simulink model "Bossi_Emanuele_EE460S3D_R99"  (R2025a)
settings: Solver=FixedStepDiscrete  StartTime=0.0  StopTime=120  FixedStep=dt0  RelTol=1e-3  EnableMultiTasking=on
PostLoadFcn:
  | %Set the size for the model
  | set_param(gcs,'Location',[10 10 1270 970])
  | %Set the zoom factor for the model
  | set_param(gcs,'ZoomFactor','100')
InitFcn:
  | tic
  | Bossi_Emanuele_EE460_Final
  | INIT_S3D_01
StartFcn:
  | tend0=toc;
  | tic;
StopFcn:
  | tend=toc;
  | disp(['Simulation time = ' num2str(tout(end)) ' sec'])
  | disp(['Real time = ' num2str(tend) ' sec'])
  | title('DONE')
  | SCORE=round((max(0,120-tout(end)-tend0))*4+10*(40-FuelBurned)+sum(100*double(PDONE)-100*double(PDONE<.5)));
  | PlotS3D(PlotInput);
  | text(15,22,['S: ' num2str(SCORE)]);
  | % Reset color scheme back to normal defaults
  | figure()
  | blkwhitebg('w');
  | close
values from neighbouring files (symbols this model uses):
  A_obs = [ 0  1  0  0  0  0 ... (first row only)    [Bossi_Emanuele_EE460_Final.m]
  B_obs = [ 0     0     0 ... (first row only)    [Bossi_Emanuele_EE460_Final.m]
  C_obs = [ 1 0 0 0 0 0 ... (first row only)    [Bossi_Emanuele_EE460_Final.m]
  d2r = pi/180    (= 0.0174532925199)    [INIT_S3D_01.m]
  D_obs = [ 0     0     0 ... (first row only)    [Bossi_Emanuele_EE460_Final.m]
  dt = 0.01    [INIT_S3D_01.m]
  dt0 = 0.001    [INIT_S3D_01.m]
  fr = 100    [INIT_S3D_01.m]
  G = [1,  1, -1, -1,  0,  0,  0,  0 ... (first row only)    [Bossi_Emanuele_EE460_Final.m]
  G_obs = eye(6)    [Bossi_Emanuele_EE460_Final.m]
  HM_S = 250    [INIT_S3D_01.m]
  HM_U = 500    [INIT_S3D_01.m]
  J = Jbase+JC0+JF+M*(Xcg^2+Ycg^2)    [INIT_S3D_01.m]
  Jbase = JC1+4*Ja+2*Ma*da^2+2*Ma*db^2    [INIT_S3D_01.m]
  JC0 = MC0/2    (= 10.2101761242)    [INIT_S3D_01.m]
  Kdtheta = 2 * zeta_th * wn_th * J_eff    [Bossi_Emanuele_EE460_Final.m]
  Kdtheta_fail = 2 * zeta_th_fail * wn_th_fail * J_eff    [Bossi_Emanuele_EE460_Final.m]
  Kdx = 2 * zeta_xy * wn_xy * M_eff    [Bossi_Emanuele_EE460_Final.m]
  Kdx_fail = 2 * zeta_xy_fail * wn_xy_fail * M_eff    [Bossi_Emanuele_EE460_Final.m]
  Kdy = 2 * zeta_xy * wn_xy * M_eff    [Bossi_Emanuele_EE460_Final.m]
  Kdy_fail = 2 * zeta_xy_fail * wn_xy_fail * M_eff    [Bossi_Emanuele_EE460_Final.m]
  Kptheta = J_eff * wn_th^2    [Bossi_Emanuele_EE460_Final.m]
  Kptheta_fail = J_eff * wn_th_fail^2    [Bossi_Emanuele_EE460_Final.m]
  Kpx = M_eff * wn_xy^2    [Bossi_Emanuele_EE460_Final.m]
  Kpx_fail = M_eff * wn_xy_fail^2    [Bossi_Emanuele_EE460_Final.m]
  Kpy = M_eff * wn_xy^2    [Bossi_Emanuele_EE460_Final.m]
  Kpy_fail = M_eff * wn_xy_fail^2    [Bossi_Emanuele_EE460_Final.m]
  L13 = sqrt(10)    [INIT_S3D_01.m]
  L24 = sqrt(6.25)    [INIT_S3D_01.m]
  LVL = LVL12    [INIT_S3D_01.m]
  M = MC+M1+M2+M3+M4+4*Ma    [INIT_S3D_01.m]
  M1 = LVL.M1    [INIT_S3D_01.m]
  M2 = LVL.M2    [INIT_S3D_01.m]
  M3 = LVL.M3    [INIT_S3D_01.m]
  M4 = LVL.M4    [INIT_S3D_01.m]
  max_qddot = [max_qddot_x; max_qddot_y; max_qddot_theta]    [Bossi_Emanuele_EE460_Final.m]
  mdti = (1/300)    (= 0.00333333333333)    [INIT_S3D_01.m]
  P = [1  1 -1 -1  0  0  0  0 ... (first row only)    [Bossi_Emanuele_EE460_Final.m]
  Pdata = [LVL.P1 LVL.P2 LVL.P3 LVL.P4]    [INIT_S3D_01.m]    (also in PlotS3D.m = R*[xt1;yt1+[0 3*tt*TV(idx-13)*TSIG(idx-13) 0]])
  PTvec = [Pdata(:,1);Pdata(:,2);Pdata(:,3);Pdata(:,4) ... (first row only)    [INIT_S3D_01.m]
  Q_obs = eye(6)    [Bossi_Emanuele_EE460_Final.m]
  r2d = 180/pi    (= 57.2957795131)    [INIT_S3D_01.m]
  r_bang = 0.5    [Bossi_Emanuele_EE460_Final.m]
  Sconfig = 1    [Bossi_Emanuele_EE460_Final.m]
  SLIM = [-100 100 ... (first row only)    [INIT_S3D_01.m]
  SQ = [.005 .01 .004 .005 .01 .004 .02 .01 .4]'    [INIT_S3D_01.m]
  SSF = 1./SQ    [INIT_S3D_01.m]
  tau = 0.5    [Bossi_Emanuele_EE460_Final.m]
  TOLdata = [LVL.P1tol LVL.P2tol LVL.P3tol LVL.P4tol]    [INIT_S3D_01.m]
  ULIM = [[Umin Umax];0 0;0 0]    [INIT_S3D_01.m]
undefined symbols (not defined in the file or in its folder): den_lp, den_lp2, DiscIntNeverNeededParam, dt1_bang_3, dt2_bang_3, dtc_bang_3, num_lp, num_lp2, q0_1
libraries: simulink x87, matrix_library x4, sl3dlib x1, aerolibutil x1, aerolibanimutils x1
(part 3 of 8)

== system Bossi_Emanuele_EE460S3D_R99/S3D_Plant/Sensors/ConvertINT16 ==
  SDouble : Inport
  Bus Creator : BusCreator  Inputs=9
  Data Type Conversion{,1..8} (9 alike) : DataTypeConversion  OutDataTypeStr=int16  SampleTime=dt0  SaturateOnIntegerOverflow=off  RndMeth=Floor
  Demux : Demux  Outputs=9
  INT16 : Outport
  wires:
  Data Type Conversion8/1 -> Bus Creator/9  "Sensor9"
  Data Type Conversion7/1 -> Bus Creator/8  "Sensor8"
  Data Type Conversion6/1 -> Bus Creator/7  "Sensor7"
  Data Type Conversion5/1 -> Bus Creator/6  "Sensor6"
  Data Type Conversion4/1 -> Bus Creator/5  "Sensor5"
  Data Type Conversion3/1 -> Bus Creator/4  "Sensor4"
  Data Type Conversion2/1 -> Bus Creator/3  "Sensor3"
  Demux/5 -> Data Type Conversion4/1
  Demux/3 -> Data Type Conversion2/1
  Demux/6 -> Data Type Conversion5/1
  Demux/4 -> Data Type Conversion3/1
  Demux/9 -> Data Type Conversion8/1
  Demux/7 -> Data Type Conversion6/1
  Demux/8 -> Data Type Conversion7/1
  SDouble/1 -> Demux/1
  Data Type Conversion1/1 -> Bus Creator/2  "Sensor2"
  Bus Creator/1 -> INT16/1  "INT16"
  Demux/1 -> Data Type Conversion/1
  Demux/2 -> Data Type Conversion1/1
  Data Type Conversion/1 -> Bus Creator/1  "Sensor1"

== system Bossi_Emanuele_EE460S3D_R99/S3D_Plant/Sensors/HealthMonitoring ==
  SensorValues : Inport
  Bus Creator1 : BusCreator  Inputs=18
  Bus Selector1 : BusSelector  OutputSignals=Sensor1,Sensor2,Sensor3,Sensor4,Sensor5,Sensor6,Sensor7,Sensor8,Sensor9
  Bus Selector2 : BusSelector  OutputSignals=Sensor1,Sensor2,Sensor3,Sensor4,Sensor5,Sensor6,Sensor7,Sensor8,Sensor9
  Subsystem : Subsystem
  Subsystem1 : Subsystem
  Subsystem2 : Subsystem
  Subsystem3 : Subsystem
  Subsystem4 : Subsystem
  Subsystem5 : Subsystem
  Subsystem6 : Subsystem
  Subsystem7 : Subsystem
  Subsystem8 : Subsystem
  Sensors : Outport
  wires:
  Bus Creator1/1 -> Sensors/1  "Sensors"
  Bus Selector2/4 -> Bus Creator1/4  "<Sensor4>"
  Bus Selector2/8 -> Bus Creator1/8  "<Sensor8>"
  Bus Selector2/6 -> Bus Creator1/6  "<Sensor6>"
  Bus Selector2/5 -> Bus Creator1/5  "<Sensor5>"
  Bus Selector2/3 -> Bus Creator1/3  "<Sensor3>"
  Bus Selector2/9 -> Bus Creator1/9  "<Sensor9>"
  Bus Selector2/2 -> Bus Creator1/2  "<Sensor2>"
  Bus Selector2/1 -> Bus Creator1/1  "<Sensor1>"
  Bus Selector2/7 -> Bus Creator1/7  "<Sensor7>"
  SensorValues/1 -> Bus Selector1/1, Bus Selector2/1
  Subsystem/1(Out1) -> Bus Creator1/10  "S1fail"
  Bus Selector1/8 -> Subsystem7/1(In1)  "<Sensor8>"
  Bus Selector1/3 -> Subsystem2/1(In1)  "<Sensor3>"
  Bus Selector1/7 -> Subsystem6/1(In1)  "<Sensor7>"
  Bus Selector1/2 -> Subsystem1/1(In1)  "<Sensor2>"
  Subsystem2/1(Out1) -> Bus Creator1/12  "S3fail"
  Subsystem1/1(Out1) -> Bus Creator1/11  "S2fail"
  Bus Selector1/6 -> Subsystem5/1(In1)  "<Sensor6>"
  Subsystem3/1(Out1) -> Bus Creator1/13  "S4fail"
  Bus Selector1/4 -> Subsystem3/1(In1)  "<Sensor4>"
  Bus Selector1/5 -> Subsystem4/1(In1)  "<Sensor5>"
  Bus Selector1/9 -> Subsystem8/1(In1)  "<Sensor9>"
  Subsystem5/1(Out1) -> Bus Creator1/15  "S6fail"
  Subsystem4/1(Out1) -> Bus Creator1/14  "S5fail"
  Subsystem6/1(Out1) -> Bus Creator1/16  "S7fail"
  Subsystem8/1(Out1) -> Bus Creator1/18  "S9fail"
  Subsystem7/1(Out1) -> Bus Creator1/17  "S8fail"
  Bus Selector1/1 -> Subsystem/1(In1)  "<Sensor1>"

== system Bossi_Emanuele_EE460S3D_R99/S3D_Plant/ThrusterValues/FailModes ==
  Ucmd : Inport
  MP : Inport  Port=2
  Bus Creator : BusCreator  Inputs=10
  Ufail1 : Subsystem  mask{Udx=1, Tank=1}
      mask prompts: Udx "Input Index of U (1-8)"; Tank "Input Fuel Tank (1-4)"
  Ufail10 : Subsystem  mask{Udx=10, Tank=1}
      mask prompts: Udx "Input Index of U (1-8)"; Tank "Input Fuel Tank (1-4)"
  Ufail2 : Subsystem  mask{Udx=2, Tank=2}
      mask prompts: Udx "Input Index of U (1-8)"; Tank "Input Fuel Tank (1-4)"
  Ufail3 : Subsystem  mask{Udx=3, Tank=3}
      mask prompts: Udx "Input Index of U (1-8)"; Tank "Input Fuel Tank (1-4)"
  Ufail4 : Subsystem  mask{Udx=4, Tank=4}
      mask prompts: Udx "Input Index of U (1-8)"; Tank "Input Fuel Tank (1-4)"
  Ufail5 : Subsystem  mask{Udx=5, Tank=1}
      mask prompts: Udx "Input Index of U (1-8)"; Tank "Input Fuel Tank (1-4)"
  Ufail6 : Subsystem  mask{Udx=6, Tank=2}
      mask prompts: Udx "Input Index of U (1-8)"; Tank "Input Fuel Tank (1-4)"
  Ufail7 : Subsystem  mask{Udx=7, Tank=3}
      mask prompts: Udx "Input Index of U (1-8)"; Tank "Input Fuel Tank (1-4)"
  Ufail8 : Subsystem  mask{Udx=8, Tank=4}
      mask prompts: Udx "Input Index of U (1-8)"; Tank "Input Fuel Tank (1-4)"
  Ufail9 : Subsystem  mask{Udx=9, Tank=1}
      mask prompts: Udx "Input Index of U (1-8)"; Tank "Input Fuel Tank (1-4)"
  U : Outport
  wires:
  Bus Creator/1 -> U/1  "U"
  Ufail7/1(Uout) -> Bus Creator/7  "U7"
  Ufail6/1(Uout) -> Bus Creator/6  "U6"
  Ufail8/1(Uout) -> Bus Creator/8  "U8"
  Ufail9/1(Uout) -> Bus Creator/9  "U9"
  Ufail10/1(Uout) -> Bus Creator/10  "U10"
  Ufail5/1(Uout) -> Bus Creator/5  "U5"
  Ufail4/1(Uout) -> Bus Creator/4  "U4"
  Ufail3/1(Uout) -> Bus Creator/3  "U3"
  Ufail2/1(Uout) -> Bus Creator/2  "U2"
  Ufail1/1(Uout) -> Bus Creator/1  "U1"
  MP/1 -> Ufail1/2(MP), Ufail3/2(MP), Ufail4/2(MP), Ufail8/2(MP), Ufail7/2(MP), Ufail6/2(MP), Ufail5/2(MP), Ufail2/2(MP)
  Ucmd/1 -> Ufail1/1(Uin), Ufail4/1(Uin), Ufail9/1(Uin), Ufail10/1(Uin), Ufail8/1(Uin), Ufail7/1(Uin), Ufail6/1(Uin), Ufail5/1(Uin), Ufail3/1(Uin), Ufail2/1(Uin)

== system Bossi_Emanuele_EE460S3D_R99/S3D_Plant/ThrusterValues/HealthMonitoring ==
  Uvalues : Inport
  UCMD : Inport  Port=2
  Bus Creator2 : BusCreator  Inputs=20
  Bus Selector10 : BusSelector  OutputSignals=U1,U2,U3,U4,U5,U6,U7,U8,U9,U10
  Bus Selector11 : BusSelector  OutputSignals=U1fail,U2fail,U3fail,U4fail,U5fail,U6fail,U7fail,U8fail,U9fail,U10fail
  DetectFailures : Subsystem
  U : Outport
  wires:
  Bus Selector10/1 -> Bus Creator2/1  "<U1>"
  Bus Selector10/2 -> Bus Creator2/2  "<U2>"
  Bus Selector10/9 -> Bus Creator2/9  "<U9>"
  Bus Selector10/5 -> Bus Creator2/5  "<U5>"
  Bus Selector10/3 -> Bus Creator2/3  "<U3>"
  Bus Selector10/6 -> Bus Creator2/6  "<U6>"
  Bus Selector10/7 -> Bus Creator2/7  "<U7>"
  Bus Selector10/8 -> Bus Creator2/8  "<U8>"
  Bus Selector10/4 -> Bus Creator2/4  "<U4>"
  Bus Selector10/10 -> Bus Creator2/10  "<U10>"
  Bus Creator2/1 -> U/1  "U"
  Bus Selector11/1 -> Bus Creator2/11  "<U1fail>"
  Bus Selector11/2 -> Bus Creator2/12  "<U2fail>"
  Bus Selector11/3 -> Bus Creator2/13  "<U3fail>"
  Bus Selector11/4 -> Bus Creator2/14  "<U4fail>"
  Bus Selector11/5 -> Bus Creator2/15  "<U5fail>"
  Bus Selector11/6 -> Bus Creator2/16  "<U6fail>"
  Bus Selector11/7 -> Bus Creator2/17  "<U7fail>"
  Bus Selector11/8 -> Bus Creator2/18  "<U8fail>"
  Bus Selector11/9 -> Bus Creator2/19  "<U9fail>"
  Bus Selector11/10 -> Bus Creator2/20  "<U10fail>"
  UCMD/1 -> DetectFailures/2(UCMD)
  Uvalues/1 -> DetectFailures/1(Uvalues), Bus Selector10/1
  DetectFailures/1(Out2) -> Bus Selector11/1

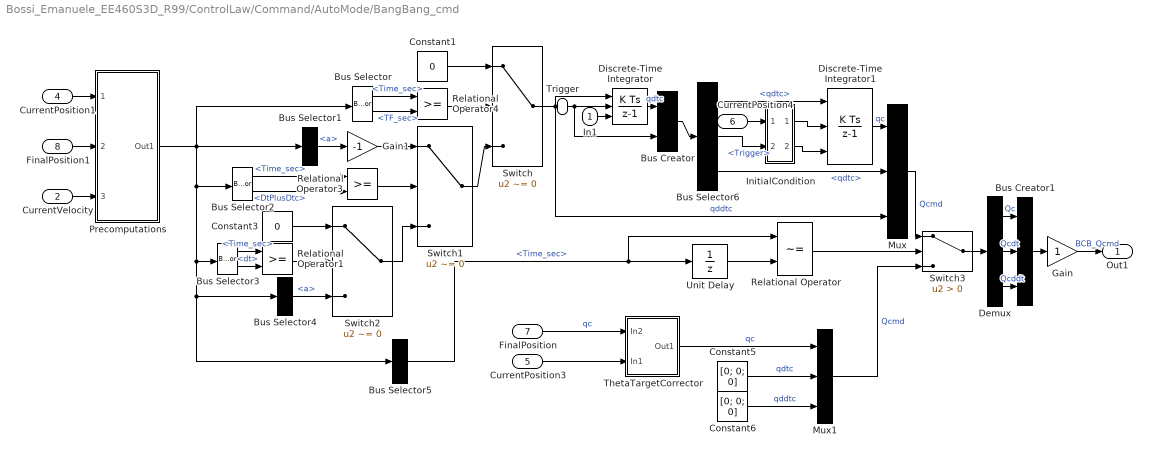
== system Bossi_Emanuele_EE460S3D_R99/ControlLaw/Command/AutoMode/BangBang_cmd ==
  In1 : Inport
  CurrentVelocity : Inport  Port=2
  Trigger : Inport  Port=3
  CurrentPosition1 : Inport  Port=4
  CurrentPosition3 : Inport  Port=5
  CurrentPosition4 : Inport  Port=6
  FinalPosition : Inport  Port=7
  FinalPosition1 : Inport  Port=8
  Bus Creator : BusCreator  Inputs=2
  Bus Creator1 : BusCreator  Inputs=3
  Bus Selector : BusSelector  OutputSignals=Time_sec,TF_sec
  Bus Selector1 : BusSelector  OutputSignals=a
  Bus Selector2 : BusSelector  OutputSignals=Time_sec,DtPlusDtc
  Bus Selector3 : BusSelector  OutputSignals=Time_sec,dt
  Bus Selector4 : BusSelector  OutputSignals=a
  Bus Selector5 : BusSelector  OutputSignals=Time_sec
  Bus Selector6 : BusSelector  OutputSignals=qdtc,Trigger,qdtc
  Constant1 : Constant  Value=0
  Constant3 : Constant  Value=0
  Constant5 : Constant  Value=[0; 0; 0]
  Constant6 : Constant  Value=[0; 0; 0]
  Demux : Demux  Outputs=3
  Discrete-Time Integrator : DiscreteIntegrator  ExternalReset=rising  InitialConditionSource=external  SampleTime=dt  ICPrevOutput=DiscIntNeverNeededParam  ICPrevScaledInput=DiscIntNeverNeededParam
  Discrete-Time Integrator1 : DiscreteIntegrator  ExternalReset=rising  InitialConditionSource=external  InitialCondition=q0_1  SampleTime=dt  ICPrevOutput=DiscIntNeverNeededParam  ICPrevScaledInput=DiscIntNeverNeededParam
  Gain : Gain
  Gain1 : Gain  Gain=-1
  InitialCondition : Subsystem
  Mux : Mux  Inputs=3
  Mux1 : Mux  Inputs=3
  Precomputations : Subsystem
  Relational Operator : RelationalOperator  Operator=~=  OutDataTypeStr=boolean  RndMeth=Simplest  InputSameDT=off
  Relational Operator1 : RelationalOperator  OutDataTypeStr=boolean  RndMeth=Simplest  InputSameDT=off
  Relational Operator3 : RelationalOperator  OutDataTypeStr=boolean  RndMeth=Simplest  InputSameDT=off
  Relational Operator4 : RelationalOperator  OutDataTypeStr=boolean  RndMeth=Simplest  InputSameDT=off
  Switch : Switch  Criteria=u2 ~= 0  Threshold=dt2_bang_3  SaturateOnIntegerOverflow=off  InputSameDT=off
  Switch1 : Switch  Criteria=u2 ~= 0  Threshold=dtc_bang_3  SaturateOnIntegerOverflow=off  InputSameDT=off
  Switch2 : Switch  Criteria=u2 ~= 0  Threshold=dt1_bang_3  SaturateOnIntegerOverflow=off  InputSameDT=off
  Switch3 : Switch  Criteria=u2 > Threshold  SaturateOnIntegerOverflow=off  InputSameDT=off
  ThetaTargetCorrector : Subsystem
  Unit Delay : UnitDelay  InitialCondition=-dt  SampleTime=dt  HasFrameUpgradeWarning=on
  Out1 : Outport
  wires:
  Bus Creator1/1 -> Gain/1
  Gain/1 -> Out1/1  "BCB_Qcmd"
  Switch3/1 -> Demux/1
  Constant5/1 -> Mux1/2  "qdtc"
  InitialCondition/2(Out2) -> Discrete-Time Integrator1/3
  Constant1/1 -> Switch/1
  Mux1/1 -> Switch3/3  "Qcmd"
  InitialCondition/1(Out1) -> Discrete-Time Integrator1/2
  Demux/1 -> Bus Creator1/1  "Qc"
  Discrete-Time Integrator1/1 -> Mux/1  "qc"
  Trigger/1 -> Discrete-Time Integrator/2, Bus Creator/2
  Unit Delay/1 -> Relational Operator/2
  Constant6/1 -> Mux1/3  "qddtc"
  Demux/2 -> Bus Creator1/2  "Qcdt"
  ThetaTargetCorrector/1(Out1) -> Mux1/1  "qc"
  Demux/3 -> Bus Creator1/3  "Qcddt"
  Switch2/1 -> Switch1/3
  Constant3/1 -> Switch2/1
  Switch/1 -> Mux/3, Discrete-Time Integrator/1  "qddtc"
  CurrentPosition4/1 -> InitialCondition/1(In1)
  FinalPosition/1 -> ThetaTargetCorrector/1(In2)  "qc"
  Bus Selector6/1 -> Discrete-Time Integrator1/1  "<qdtc>"
  Mux/1 -> Switch3/1  "Qcmd"
  Relational Operator/1 -> Switch3/2
  Switch1/1 -> Switch/3
  CurrentPosition3/1 -> ThetaTargetCorrector/2(In1)
  CurrentPosition1/1 -> Precomputations/1(CurrentPosition1)
  FinalPosition1/1 -> Precomputations/2(FinalPosition1)
  Precomputations/1(Out1) -> Bus Selector/1, Bus Selector2/1, Bus Selector5/1, Bus Selector4/1, Bus Selector3/1, Bus Selector1/1
  Gain1/1 -> Switch1/1
  Relational Operator1/1 -> Switch2/2
  Relational Operator3/1 -> Switch1/2
  Relational Operator4/1 -> Switch/2
  Bus Selector1/1 -> Gain1/1  "<a>"
  Bus Selector2/1 -> Relational Operator3/1  "<Time_sec>"
  Bus Selector2/2 -> Relational Operator3/2  "<DtPlusDtc>"
  Bus Selector3/2 -> Relational Operator1/2  "<dt>"
  Bus Selector3/1 -> Relational Operator1/1  "<Time_sec>"
  Bus Selector4/1 -> Switch2/3  "<a>"
  Bus Selector5/1 -> Relational Operator/1, Unit Delay/1  "<Time_sec>"
  Bus Selector/1 -> Relational Operator4/1  "<Time_sec>"
  Bus Selector/2 -> Relational Operator4/2  "<TF_sec>"
  Discrete-Time Integrator/1 -> Bus Creator/1  "qdtc"
  Bus Creator/1 -> Bus Selector6/1
  Bus Selector6/2 -> InitialCondition/2(In2)  "<Trigger>"
  Bus Selector6/3 -> Mux/2  "<qdtc>"
  In1/1 -> Discrete-Time Integrator/3
  CurrentVelocity/1 -> Precomputations/3(CurrentVelocity)

== system Bossi_Emanuele_EE460S3D_R99/ControlLaw/Command/AutoMode/FinalPositionSelector ==
  In2 : Inport
  If : If  IfExpression=u1 < 1.5  ElseIfExpressions=u1 < 2.5,u1 < 3.5
  Merge : Merge  Inputs=4
  Pdata1 : Subsystem  TreatAsAtomicUnit=on
  Pdata2 : Subsystem  TreatAsAtomicUnit=on
  Pdata3 : Subsystem  TreatAsAtomicUnit=on
  Pdata4 : Subsystem  TreatAsAtomicUnit=on
  FinalPosition : Outport
  wires:
  In2/1 -> If/1
  If/1 -> Pdata1/Action
  Pdata1/1(Out1) -> Merge/1
  Pdata2/1(Out1) -> Merge/2
  Pdata3/1(Out1) -> Merge/3
  Pdata4/1(Out1) -> Merge/4
  If/2 -> Pdata2/Action
  If/3 -> Pdata3/Action
  If/4 -> Pdata4/Action
  Merge/1 -> FinalPosition/1  "FinalPosition"

== system Bossi_Emanuele_EE460S3D_R99/ControlLaw/Command/AutoMode/PositionTrigger ==
  In1 : Inport
  Trigger : TriggerPort  VariantControl=(inherit)
  Bus Selector : BusSelector  OutputSignals=Xpos_m,Ypos_m,theta_pos_deg
  Vector Concatenate : Concatenate  NumInputs=3
  CurrentPosition1 : Outport
  wires:
  Bus Selector/1 -> Vector Concatenate/1  "<Xpos_m>"
  In1/1 -> Bus Selector/1
  Bus Selector/2 -> Vector Concatenate/2  "<Ypos_m>"
  Bus Selector/3 -> Vector Concatenate/3  "<theta_pos_deg>"
  Vector Concatenate/1 -> CurrentPosition1/1  "TriggeredPosition"

== system Bossi_Emanuele_EE460S3D_R99/ControlLaw/Command/AutoMode/TriggerCondition ==
  In2 : Inport
  Relational Operator : RelationalOperator  Operator=~=  OutDataTypeStr=boolean  RndMeth=Simplest  InputSameDT=off
  Unit Delay : UnitDelay  SampleTime=dt  HasFrameUpgradeWarning=on
  Trigger : Outport
  wires:
  Relational Operator/1 -> Trigger/1  "Trigger"
  In2/1 -> Relational Operator/1, Unit Delay/1
  Unit Delay/1 -> Relational Operator/2

== system Bossi_Emanuele_EE460S3D_R99/ControlLaw/Command/AutoMode/VelocityTrigger ==
  In1 : Inport
  Trigger : TriggerPort  VariantControl=(inherit)
  Bus Selector : BusSelector  OutputSignals=Xvel_mps,Yvel_mps,theta_vel_degps
  Vector Concatenate : Concatenate  NumInputs=3
  CurrentVelocity : Outport
  wires:
  In1/1 -> Bus Selector/1
  Vector Concatenate/1 -> CurrentVelocity/1  "TriggeredVelocity"
  Bus Selector/1 -> Vector Concatenate/1  "<Xvel_mps>"
  Bus Selector/2 -> Vector Concatenate/2  "<Yvel_mps>"
  Bus Selector/3 -> Vector Concatenate/3  "<theta_vel_degps>"

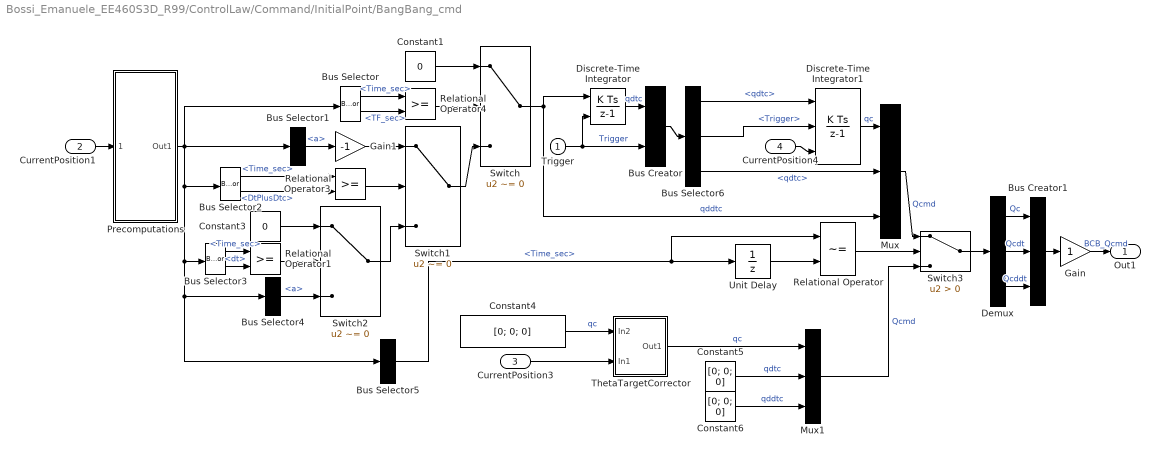
== system Bossi_Emanuele_EE460S3D_R99/ControlLaw/Command/InitialPoint/BangBang_cmd ==
  Trigger : Inport
  CurrentPosition1 : Inport  Port=2
  CurrentPosition3 : Inport  Port=3
  CurrentPosition4 : Inport  Port=4
  Bus Creator : BusCreator  Inputs=2
  Bus Creator1 : BusCreator  Inputs=3
  Bus Selector : BusSelector  OutputSignals=Time_sec,TF_sec
  Bus Selector1 : BusSelector  OutputSignals=a
  Bus Selector2 : BusSelector  OutputSignals=Time_sec,DtPlusDtc
  Bus Selector3 : BusSelector  OutputSignals=Time_sec,dt
  Bus Selector4 : BusSelector  OutputSignals=a
  Bus Selector5 : BusSelector  OutputSignals=Time_sec
  Bus Selector6 : BusSelector  OutputSignals=qdtc,Trigger,qdtc
  Constant1 : Constant  Value=0
  Constant3 : Constant  Value=0
  Constant4 : Constant  Value=[0; 0; 0]  SampleTime=dt
  Constant5 : Constant  Value=[0; 0; 0]
  Constant6 : Constant  Value=[0; 0; 0]
  Demux : Demux  Outputs=3
  Discrete-Time Integrator : DiscreteIntegrator  ExternalReset=rising  SampleTime=dt  ICPrevOutput=DiscIntNeverNeededParam  ICPrevScaledInput=DiscIntNeverNeededParam
  Discrete-Time Integrator1 : DiscreteIntegrator  ExternalReset=rising  InitialConditionSource=external  InitialCondition=q0_1  SampleTime=dt  ICPrevOutput=DiscIntNeverNeededParam  ICPrevScaledInput=DiscIntNeverNeededParam
  Gain : Gain
  Gain1 : Gain  Gain=-1
  Mux : Mux  Inputs=3
  Mux1 : Mux  Inputs=3
  Precomputations : Subsystem
  Relational Operator : RelationalOperator  Operator=~=  OutDataTypeStr=boolean  RndMeth=Simplest  InputSameDT=off
  Relational Operator1 : RelationalOperator  OutDataTypeStr=boolean  RndMeth=Simplest  InputSameDT=off
  Relational Operator3 : RelationalOperator  OutDataTypeStr=boolean  RndMeth=Simplest  InputSameDT=off
  Relational Operator4 : RelationalOperator  OutDataTypeStr=boolean  RndMeth=Simplest  InputSameDT=off
  Switch : Switch  Criteria=u2 ~= 0  Threshold=dt2_bang_3  SaturateOnIntegerOverflow=off  InputSameDT=off
  Switch1 : Switch  Criteria=u2 ~= 0  Threshold=dtc_bang_3  SaturateOnIntegerOverflow=off  InputSameDT=off
  Switch2 : Switch  Criteria=u2 ~= 0  Threshold=dt1_bang_3  SaturateOnIntegerOverflow=off  InputSameDT=off
  Switch3 : Switch  Criteria=u2 > Threshold  SaturateOnIntegerOverflow=off  InputSameDT=off
  ThetaTargetCorrector : Subsystem
  Unit Delay : UnitDelay  InitialCondition=-dt  SampleTime=dt  HasFrameUpgradeWarning=on
  Out1 : Outport
  wires:
  Bus Creator1/1 -> Gain/1
  Gain/1 -> Out1/1  "BCB_Qcmd"
  Switch3/1 -> Demux/1
  Constant5/1 -> Mux1/2  "qdtc"
  Constant1/1 -> Switch/1
  Mux1/1 -> Switch3/3  "Qcmd"
  Demux/1 -> Bus Creator1/1  "Qc"
  Discrete-Time Integrator1/1 -> Mux/1  "qc"
  Unit Delay/1 -> Relational Operator/2
  Constant6/1 -> Mux1/3  "qddtc"
  Demux/2 -> Bus Creator1/2  "Qcdt"
  ThetaTargetCorrector/1(Out1) -> Mux1/1  "qc"
  Demux/3 -> Bus Creator1/3  "Qcddt"
  Switch2/1 -> Switch1/3
  Constant3/1 -> Switch2/1
  Switch/1 -> Mux/3, Discrete-Time Integrator/1  "qddtc"
  CurrentPosition4/1 -> Discrete-Time Integrator1/3
  Constant4/1 -> ThetaTargetCorrector/1(In2)  "qc"
  Bus Selector6/1 -> Discrete-Time Integrator1/1  "<qdtc>"
  Mux/1 -> Switch3/1  "Qcmd"
  Relational Operator/1 -> Switch3/2
  Switch1/1 -> Switch/3
  CurrentPosition3/1 -> ThetaTargetCorrector/2(In1)
  CurrentPosition1/1 -> Precomputations/1(CurrentPosition1)
  Precomputations/1(Out1) -> Bus Selector/1, Bus Selector2/1, Bus Selector5/1, Bus Selector4/1, Bus Selector3/1, Bus Selector1/1
  Gain1/1 -> Switch1/1
  Relational Operator1/1 -> Switch2/2
  Relational Operator3/1 -> Switch1/2
  Relational Operator4/1 -> Switch/2
  Bus Selector1/1 -> Gain1/1  "<a>"
  Bus Selector2/1 -> Relational Operator3/1  "<Time_sec>"
  Bus Selector2/2 -> Relational Operator3/2  "<DtPlusDtc>"
  Bus Selector3/2 -> Relational Operator1/2  "<dt>"
  Bus Selector3/1 -> Relational Operator1/1  "<Time_sec>"
  Bus Selector4/1 -> Switch2/3  "<a>"
  Bus Selector5/1 -> Relational Operator/1, Unit Delay/1  "<Time_sec>"
  Bus Selector/1 -> Relational Operator4/1  "<Time_sec>"
  Bus Selector/2 -> Relational Operator4/2  "<TF_sec>"
  Discrete-Time Integrator/1 -> Bus Creator/1  "qdtc"
  Bus Creator/1 -> Bus Selector6/1
  Bus Selector6/3 -> Mux/2  "<qdtc>"
  Trigger/1 -> Discrete-Time Integrator/2, Bus Creator/2  "Trigger"
  Bus Selector6/2 -> Discrete-Time Integrator1/2  "<Trigger>"

== system Bossi_Emanuele_EE460S3D_R99/ControlLaw/Command/Joystick/Hold ==
  In1 : Inport
  Logical Operator : Logic  Operator=NOT  AllPortsSameDT=off  OutDataTypeStr=boolean
  Logical Operator1 : Logic  AllPortsSameDT=off  OutDataTypeStr=boolean
  Logical Operator2 : Logic  Operator=NOT  AllPortsSameDT=off  OutDataTypeStr=boolean
  Switch : Switch  Criteria=u2 > Threshold  SaturateOnIntegerOverflow=off  InputSameDT=off
  Unit Delay : UnitDelay  SampleTime=-1  HasFrameUpgradeWarning=on
  Unit Delay1 : UnitDelay  SampleTime=dt  HasFrameUpgradeWarning=on
  Unit Delay2 : UnitDelay  SampleTime=dt  HasFrameUpgradeWarning=on
  Out1 : Outport
  wires:
  Logical Operator2/1 -> Switch/1
  Switch/1 -> Out1/1, Unit Delay2/1, Unit Delay1/1  "ManualMode"
  Unit Delay1/1 -> Switch/3
  Unit Delay2/1 -> Logical Operator2/1
  Unit Delay/1 -> Logical Operator/1
  Logical Operator1/1 -> Switch/2  "pressEvent"
  Logical Operator/1 -> Logical Operator1/2  "NOT_prevButton"
  In1/1 -> Unit Delay/1, Logical Operator1/1  "Button"

== system Bossi_Emanuele_EE460S3D_R99/ControlLaw/Command/Joystick/Hold1 ==
  In1 : Inport
  Logical Operator : Logic  Operator=NOT  AllPortsSameDT=off  OutDataTypeStr=boolean
  Logical Operator1 : Logic  AllPortsSameDT=off  OutDataTypeStr=boolean
  Logical Operator2 : Logic  Operator=NOT  AllPortsSameDT=off  OutDataTypeStr=boolean
  Switch : Switch  Criteria=u2 > Threshold  SaturateOnIntegerOverflow=off  InputSameDT=off
  Unit Delay : UnitDelay  SampleTime=-1  HasFrameUpgradeWarning=on
  Unit Delay1 : UnitDelay  SampleTime=dt  HasFrameUpgradeWarning=on
  Unit Delay2 : UnitDelay  SampleTime=dt  HasFrameUpgradeWarning=on
  Out1 : Outport
  wires:
  Logical Operator2/1 -> Switch/1
  Switch/1 -> Out1/1, Unit Delay2/1, Unit Delay1/1  "AutoON"
  Unit Delay1/1 -> Switch/3
  Unit Delay2/1 -> Logical Operator2/1
  Unit Delay/1 -> Logical Operator/1
  Logical Operator1/1 -> Switch/2  "pressEvent"
  Logical Operator/1 -> Logical Operator1/2  "NOT_prevButton"
  In1/1 -> Unit Delay/1, Logical Operator1/1  "Button"

== system Bossi_Emanuele_EE460S3D_R99/ControlLaw/Command/Joystick/MissionNum ==
  In1 : Inport
  In2 : Inport  Port=2
  In3 : Inport  Port=3
  In4 : Inport  Port=4
  Data Type Conversion{,1..3} (4 alike) : DataTypeConversion  OutDataTypeStr=double  SaturateOnIntegerOverflow=off  RndMeth=Floor
  Gain : Gain
  Gain1 : Gain  Gain=2
  Gain2 : Gain  Gain=3
  Gain3 : Gain  Gain=4
  Sum : Sum  Inputs=++++
  Out1 : Outport
  wires:
  In3/1 -> Data Type Conversion2/1
  Gain3/1 -> Sum/4
  Data Type Conversion2/1 -> Gain2/1
  Gain1/1 -> Sum/2
  In4/1 -> Data Type Conversion3/1
  Gain2/1 -> Sum/3
  In2/1 -> Data Type Conversion1/1
  Gain/1 -> Sum/1
  Data Type Conversion3/1 -> Gain3/1
  Data Type Conversion/1 -> Gain/1
  In1/1 -> Data Type Conversion/1
  Data Type Conversion1/1 -> Gain1/1
  Sum/1 -> Out1/1  "MissionNum"

== system Bossi_Emanuele_EE460S3D_R99/ControlLaw/Command/Joystick/PointToGo ==
  Y_IN : Inport
  In1 : Inport  Port=2
  Bus Creator : BusCreator  Inputs=3
  Bus Creator1 : BusCreator  Inputs=4
  Bus Selector : BusSelector  OutputSignals=P1Done,P2Done,P3Done,P4Done
  Bus Selector1 : BusSelector  OutputSignals=UserChoice,MissionNum
  Bus Selector2 : BusSelector  OutputSignals=UserChoice,newSelection
  Bus Selector3 : BusSelector  OutputSignals=hold_active,MissionNum
  Cast To Double : DataTypeConversion  OutDataTypeStr=double  SaturateOnIntegerOverflow=off  RndMeth=Floor
  Compare To Constant : simulink/Logic and Bit Operations/Compare To Constant  relop=<  const=1  OutDataTypeStr=boolean
  Constant : Constant
  Data Type Conversion{,1..3} (4 alike) : DataTypeConversion  OutDataTypeStr=double  SaturateOnIntegerOverflow=off  RndMeth=Floor
  Hold : Subsystem
  Sum : Sum  Inputs=++++
  Sum2 : Sum  Inputs=|++
  Switch : Switch  Criteria=u2 > Threshold  Threshold=0.5  SaturateOnIntegerOverflow=off  InputSameDT=off
  Switch1 : Switch  Criteria=u2 > Threshold  SaturateOnIntegerOverflow=off  InputSameDT=off
  Unit Delay : UnitDelay  InitialCondition=1  SampleTime=dt  HasFrameUpgradeWarning=on
  Out1 : Outport
  wires:
  In1/1 -> Bus Creator/3, Compare To Constant/1
  Bus Selector/1 -> Data Type Conversion/1  "<P1Done>"
  Data Type Conversion1/1 -> Sum/2
  Bus Selector/4 -> Data Type Conversion3/1  "<P4Done>"
  Y_IN/1 -> Bus Selector/1
  Bus Selector/3 -> Data Type Conversion2/1  "<P3Done>"
  Data Type Conversion2/1 -> Sum/3
  Bus Selector/2 -> Data Type Conversion1/1  "<P2Done>"
  Compare To Constant/1 -> Bus Creator/2  "SwitchCondition"
  Data Type Conversion/1 -> Sum/1
  Data Type Conversion3/1 -> Sum/4
  Sum/1 -> Sum2/1
  Sum2/1 -> Bus Creator/1  "MissionNum"
  Constant/1 -> Sum2/2
  Bus Creator/1 -> Bus Selector1/1, Hold/1(In1)  "Trigger"
  Unit Delay/1 -> Switch/3  "UserChoice_latched_prev"
  Switch/1 -> Unit Delay/1, Cast To Double/1  "UserChoice_latched"
  Bus Selector1/1 -> Bus Creator1/1  "<UserChoice>"
  Bus Creator1/1 -> Bus Selector2/1, Bus Selector3/1
  Bus Selector2/1 -> Switch/1  "<UserChoice>"
  Bus Selector2/2 -> Switch/2  "<newSelection>"
  Bus Selector3/1 -> Switch1/2  "<hold_active>"
  Switch1/1 -> Out1/1  "PointToGo"
  Hold/2(Out2) -> Bus Creator1/4
  Hold/1(Out1) -> Bus Creator1/3
  Bus Selector1/2 -> Bus Creator1/2  "<MissionNum>"
  Bus Selector3/2 -> Switch1/3  "<MissionNum>"
  Cast To Double/1 -> Switch1/1

== system Bossi_Emanuele_EE460S3D_R99/ControlLaw/Command/ManualMode/Theta_cmd ==
  In1 : Inport
  In4 : Inport  Port=2
  In3 : Inport  Port=3
  In2 : Inport  Port=4
  In5 : Inport  Port=5
  Bus Creator5 : BusCreator  Inputs=1
  Bus Creator6 : BusCreator  Inputs=1
  Bus Selector5 : BusSelector  OutputSignals=theta_ddot_cmd,theta_ddot_cmd
  Bus Selector6 : BusSelector  OutputSignals=theta_dot_cmd,theta_dot_cmd,theta_dot_cmd
  Constant2 : Constant  Value=3
  Dead Zone2 : DeadZone  LowerValue=-0.05  UpperValue=0.05
  Discrete-Time Integrator4 : DiscreteIntegrator  ExternalReset=either  InitialConditionSource=external  SampleTime=dt  ICPrevOutput=DiscIntNeverNeededParam  ICPrevScaledInput=DiscIntNeverNeededParam
  Discrete-Time Integrator5 : DiscreteIntegrator  ExternalReset=either  InitialConditionSource=external  SampleTime=dt  ICPrevOutput=DiscIntNeverNeededParam  ICPrevScaledInput=DiscIntNeverNeededParam
  Gain : Gain  Gain=-1
  Gain2 : Gain  Gain=20
  Gain5 : Gain  Gain=1/tau
  Math Function2 : Math  Operator=pow
  Saturation : Saturate  UpperLimit=800  LowerLimit=-800
  Sum2 : Sum  Inputs=|-+|
  Out1 : Outport
  Out2 : Outport  Port=2
  Out3 : Outport  Port=3
  wires:
  Discrete-Time Integrator5/1 -> Out1/1  "theta_cmd"
  Bus Selector6/3 -> Out2/1  "<theta_dot_cmd>"
  Bus Selector5/2 -> Out3/1  "<theta_ddot_cmd>"
  Gain5/1 -> Bus Creator5/1  "theta_ddot_cmd"
  In1/1 -> Saturation/1
  Dead Zone2/1 -> Math Function2/1  "u_r_f"
  Constant2/1 -> Math Function2/2
  Bus Creator6/1 -> Bus Selector6/1
  Math Function2/1 -> Gain2/1  "u_r_shaped"
  Bus Selector6/2 -> Discrete-Time Integrator5/1  "<theta_dot_cmd>"
  Bus Selector5/1 -> Discrete-Time Integrator4/1  "<theta_ddot_cmd>"
  Gain2/1 -> Sum2/2  "theta_dot_des"
  Bus Selector6/1 -> Sum2/1  "<theta_dot_cmd>"
  Discrete-Time Integrator4/1 -> Bus Creator6/1  "theta_dot_cmd"
  Sum2/1 -> Gain5/1
  Bus Creator5/1 -> Bus Selector5/1
  Gain/1 -> Dead Zone2/1
  Saturation/1 -> Gain/1
  In3/1 -> Discrete-Time Integrator4/3
  In2/1 -> Discrete-Time Integrator4/2
  In4/1 -> Discrete-Time Integrator5/3
  In5/1 -> Discrete-Time Integrator5/2

== system Bossi_Emanuele_EE460S3D_R99/ControlLaw/Command/ManualMode/X_cmd ==
  In1 : Inport
  In5 : Inport  Port=2
  In3 : Inport  Port=3
  In2 : Inport  Port=4
  In4 : Inport  Port=5
  Bus Creator1 : BusCreator  Inputs=1
  Bus Creator2 : BusCreator  Inputs=1
  Bus Selector1 : BusSelector  OutputSignals=xddot_cmd,xddot_cmd
  Bus Selector2 : BusSelector  OutputSignals=xdot_cmd,xdot_cmd,xdot_cmd
  Constant : Constant  Value=3
  Dead Zone : DeadZone  LowerValue=-0.05  UpperValue=0.05
  Discrete-Time Integrator : DiscreteIntegrator  ExternalReset=either  InitialConditionSource=external  SampleTime=dt  ICPrevOutput=DiscIntNeverNeededParam  ICPrevScaledInput=DiscIntNeverNeededParam
  Discrete-Time Integrator1 : DiscreteIntegrator  ExternalReset=either  InitialConditionSource=external  SampleTime=dt  ICPrevOutput=DiscIntNeverNeededParam  ICPrevScaledInput=DiscIntNeverNeededParam
  Gain : Gain  Gain=4
  Gain3 : Gain  Gain=1/tau
  Math Function : Math  Operator=pow
  Saturation : Saturate  UpperLimit=200  LowerLimit=-200
  Sum : Sum  Inputs=|-+|
  Out1 : Outport
  Out2 : Outport  Port=2
  Out3 : Outport  Port=3
  wires:
  Bus Selector2/2 -> Discrete-Time Integrator1/1  "<xdot_cmd>"
  Discrete-Time Integrator1/1 -> Out1/1  "x_cmd"
  Gain3/1 -> Bus Creator1/1  "xddot_cmd"
  Bus Selector2/3 -> Out2/1  "<xdot_cmd>"
  Bus Selector2/1 -> Sum/1  "<xdot_cmd>"
  Bus Creator2/1 -> Bus Selector2/1
  Dead Zone/1 -> Math Function/1  "u_x_f"
  Bus Selector1/2 -> Out3/1  "<xddot_cmd>"
  Gain/1 -> Sum/2  "xdot_des"
  Bus Creator1/1 -> Bus Selector1/1
  In1/1 -> Saturation/1
  Discrete-Time Integrator/1 -> Bus Creator2/1  "xdot_cmd"
  Sum/1 -> Gain3/1
  Bus Selector1/1 -> Discrete-Time Integrator/1  "<xddot_cmd>"
  Constant/1 -> Math Function/2
  Math Function/1 -> Gain/1  "u_x_shaped"
  Saturation/1 -> Dead Zone/1
  In2/1 -> Discrete-Time Integrator/2
  In3/1 -> Discrete-Time Integrator/3
  In4/1 -> Discrete-Time Integrator1/2
  In5/1 -> Discrete-Time Integrator1/3

== system Bossi_Emanuele_EE460S3D_R99/ControlLaw/Command/ManualMode/Y_cmd ==
  In1 : Inport
  In4 : Inport  Port=2
  In3 : Inport  Port=3
  In2 : Inport  Port=4
  In5 : Inport  Port=5
  Bus Creator3 : BusCreator  Inputs=1
  Bus Creator4 : BusCreator  Inputs=1
  Bus Selector3 : BusSelector  OutputSignals=yddot_cmd,yddot_cmd
  Bus Selector4 : BusSelector  OutputSignals=ydot_cmd,ydot_cmd,ydot_cmd
  Constant1 : Constant  Value=3
  Dead Zone1 : DeadZone  LowerValue=-0.05  UpperValue=0.05
  Discrete-Time Integrator2 : DiscreteIntegrator  ExternalReset=either  InitialConditionSource=external  SampleTime=dt  ICPrevOutput=DiscIntNeverNeededParam  ICPrevScaledInput=DiscIntNeverNeededParam
  Discrete-Time Integrator3 : DiscreteIntegrator  ExternalReset=either  InitialConditionSource=external  SampleTime=dt  ICPrevOutput=DiscIntNeverNeededParam  ICPrevScaledInput=DiscIntNeverNeededParam
  Gain : Gain  Gain=-1
  Gain1 : Gain  Gain=4
  Gain4 : Gain  Gain=1/tau
  Math Function1 : Math  Operator=pow
  Saturation : Saturate  UpperLimit=200  LowerLimit=-200
  Sum1 : Sum  Inputs=|-+|
  Out1 : Outport
  Out2 : Outport  Port=2
  Out3 : Outport  Port=3
  wires:
  Bus Selector4/3 -> Out2/1  "<ydot_cmd>"
  Discrete-Time Integrator3/1 -> Out1/1  "y_cmd"
  Bus Selector3/2 -> Out3/1  "<yddot_cmd>"
  Constant1/1 -> Math Function1/2
  Dead Zone1/1 -> Math Function1/1  "u_y_f"
  In1/1 -> Saturation/1
  Gain4/1 -> Bus Creator3/1  "yddot_cmd"
  Bus Selector3/1 -> Discrete-Time Integrator2/1  "<yddot_cmd>"
  Sum1/1 -> Gain4/1
  Bus Selector4/2 -> Discrete-Time Integrator3/1  "<ydot_cmd>"
  Bus Creator3/1 -> Bus Selector3/1
  Bus Creator4/1 -> Bus Selector4/1
  Discrete-Time Integrator2/1 -> Bus Creator4/1  "ydot_cmd"
  Gain1/1 -> Sum1/2  "ydot_des"
  Math Function1/1 -> Gain1/1  "u_y_shaped"
  Bus Selector4/1 -> Sum1/1  "<ydot_cmd>"
  Gain/1 -> Dead Zone1/1
  Saturation/1 -> Gain/1
  In3/1 -> Discrete-Time Integrator2/3
  In2/1 -> Discrete-Time Integrator2/2
  In4/1 -> Discrete-Time Integrator3/3
  In5/1 -> Discrete-Time Integrator3/2

== system Bossi_Emanuele_EE460S3D_R99/ControlLaw/Command/Trigger1/PositionTrigger ==
  In1 : Inport
  Trigger : TriggerPort  TriggerType=either  VariantControl=(inherit)
  Bus Selector : BusSelector  OutputSignals=Xpos_m,Ypos_m,theta_pos_deg
  Vector Concatenate : Concatenate  NumInputs=3
  CurrentPosition1 : Outport
  wires:
  Bus Selector/1 -> Vector Concatenate/1  "<Xpos_m>"
  In1/1 -> Bus Selector/1
  Bus Selector/2 -> Vector Concatenate/2  "<Ypos_m>"
  Bus Selector/3 -> Vector Concatenate/3  "<theta_pos_deg>"
  Vector Concatenate/1 -> CurrentPosition1/1  "TriggeredPosition"

== system Bossi_Emanuele_EE460S3D_R99/ControlLaw/Command/Trigger1/TriggerCondition ==
  In2 : Inport
  Relational Operator : RelationalOperator  Operator=~=  OutDataTypeStr=boolean  RndMeth=Simplest  InputSameDT=off
  Unit Delay : UnitDelay  SampleTime=dt  HasFrameUpgradeWarning=on
  Trigger : Outport
  wires:
  Relational Operator/1 -> Trigger/1  "Trigger"
  In2/1 -> Relational Operator/1, Unit Delay/1
  Unit Delay/1 -> Relational Operator/2

== system Bossi_Emanuele_EE460S3D_R99/ControlLaw/Command/Trigger2/PositionTrigger ==
  In1 : Inport
  Trigger : TriggerPort  TriggerType=either  VariantControl=(inherit)
  Bus Selector : BusSelector  OutputSignals=Xpos_m,Ypos_m,theta_pos_deg
  Vector Concatenate : Concatenate  NumInputs=3
  CurrentPosition1 : Outport
  wires:
  Bus Selector/1 -> Vector Concatenate/1  "<Xpos_m>"
  In1/1 -> Bus Selector/1
  Bus Selector/2 -> Vector Concatenate/2  "<Ypos_m>"
  Bus Selector/3 -> Vector Concatenate/3  "<theta_pos_deg>"
  Vector Concatenate/1 -> CurrentPosition1/1  "TriggeredPosition"

== system Bossi_Emanuele_EE460S3D_R99/ControlLaw/Command/Trigger2/TriggerCondition ==
  In2 : Inport
  Relational Operator : RelationalOperator  Operator=~=  OutDataTypeStr=boolean  RndMeth=Simplest  InputSameDT=off
  Unit Delay : UnitDelay  SampleTime=dt  HasFrameUpgradeWarning=on
  Trigger : Outport
  wires:
  Relational Operator/1 -> Trigger/1  "Trigger"
  In2/1 -> Relational Operator/1, Unit Delay/1
  Unit Delay/1 -> Relational Operator/2

== system Bossi_Emanuele_EE460S3D_R99/ControlLaw/Command/Trigger2/VelocityTrigger ==
  In1 : Inport
  Trigger : TriggerPort  TriggerType=either  VariantControl=(inherit)
  Bus Selector : BusSelector  OutputSignals=Xvel_mps,Yvel_mps,theta_vel_degps
  Vector Concatenate : Concatenate  NumInputs=3
  CurrentVelocity : Outport
  wires:
  In1/1 -> Bus Selector/1
  Vector Concatenate/1 -> CurrentVelocity/1  "TriggeredVelocity"
  Bus Selector/1 -> Vector Concatenate/1  "<Xvel_mps>"
  Bus Selector/2 -> Vector Concatenate/2  "<Yvel_mps>"
  Bus Selector/3 -> Vector Concatenate/3  "<theta_vel_degps>"

== system Bossi_Emanuele_EE460S3D_R99/ControlLaw/ControlAllocation/A/WTI ==
  Y_IN : Inport
  Bus Selector : BusSelector  OutputSignals=U1fail,U2fail,U3fail,U4fail,U5fail,U6fail,U7fail,U8fail
  Constant{,1..7} (8 alike) : Constant
  Constant8 : Constant  Value=[0.000001 0.000001 0.000001 0.000001 0.000001 0.000001 0.000001 0.000001]  SampleTime=dt
  Create Diagonal Matrix : matrix_library/Create Diagonal Matrix
      settings: LibrarySourceBlock=|
      | simulink/Matrix
      | Operations/Create Diagonal
      | Matrix
  Create Diagonal Matrix1 : matrix_library/Create Diagonal Matrix
      settings: LibrarySourceBlock=|
      | simulink/Matrix
      | Operations/Create Diagonal
      | Matrix
  Sum{,1..7} (8 alike) : Sum  Inputs=|-+
  Switch : Switch  Criteria=u2 > Threshold  SaturateOnIntegerOverflow=off  InputSameDT=off
  Vector Concatenate : Concatenate  NumInputs=8
  Out1 : Outport
  wires:
  Y_IN/1 -> Bus Selector/1  "Y_IN"
  Constant/1 -> Sum/2
  Constant1/1 -> Sum1/2
  Constant2/1 -> Sum2/2
  Constant3/1 -> Sum3/2
  Constant4/1 -> Sum4/2
  Constant5/1 -> Sum5/2
  Constant6/1 -> Sum6/2
  Constant7/1 -> Sum7/2
  Sum/1 -> Vector Concatenate/1
  Sum1/1 -> Vector Concatenate/2
  Sum2/1 -> Vector Concatenate/3
  Sum3/1 -> Vector Concatenate/4
  Sum4/1 -> Vector Concatenate/5
  Sum5/1 -> Vector Concatenate/6
  Sum6/1 -> Vector Concatenate/7
  Sum7/1 -> Vector Concatenate/8
  Vector Concatenate/1 -> Create Diagonal Matrix/1
  Switch/1 -> Out1/1  "WTI"
  Bus Selector/1 -> Sum/1  "<U1fail>"
  Bus Selector/2 -> Sum1/1  "<U2fail>"
  Bus Selector/3 -> Sum2/1  "<U3fail>"
  Bus Selector/4 -> Sum3/1  "<U4fail>"
  Bus Selector/5 -> Sum4/1  "<U5fail>"
  Bus Selector/6 -> Sum5/1  "<U6fail>"
  Bus Selector/7 -> Sum6/1  "<U7fail>"
  Bus Selector/8 -> Sum7/1  "<U8fail>"
  Create Diagonal Matrix/1 -> Switch/1, Switch/2  "WTI"
  Constant8/1 -> Create Diagonal Matrix1/1
  Create Diagonal Matrix1/1 -> Switch/3

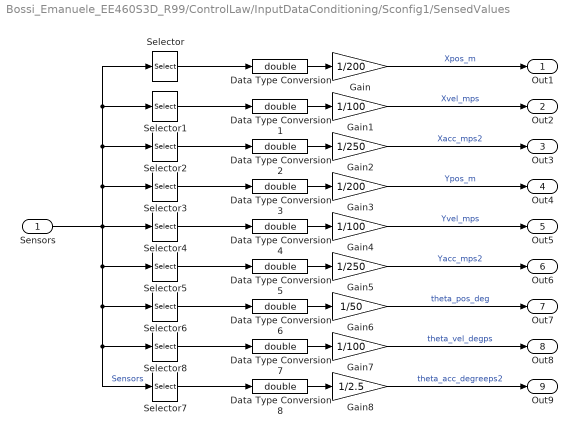
== system Bossi_Emanuele_EE460S3D_R99/ControlLaw/InputDataConditioning/Sconfig1/SensedValues ==
  Sensors : Inport
  Data Type Conversion{,1..8} (9 alike) : DataTypeConversion  OutDataTypeStr=double  SaturateOnIntegerOverflow=off  RndMeth=Floor
  Gain : Gain  Gain=1/200
  Gain1 : Gain  Gain=1/100
  Gain2 : Gain  Gain=1/250
  Gain3 : Gain  Gain=1/200
  Gain4 : Gain  Gain=1/100
  Gain5 : Gain  Gain=1/250
  Gain6 : Gain  Gain=1/50
  Gain7 : Gain  Gain=1/100
  Gain8 : Gain  Gain=1/2.5
  Selector : Selector  InputPortWidth=9  IndexOptions=Index vector (dialog)  Indices=1  OutputSizes=1
  Selector1 : Selector  InputPortWidth=9  IndexOptions=Index vector (dialog)  Indices=2  OutputSizes=1
  Selector2 : Selector  InputPortWidth=9  IndexOptions=Index vector (dialog)  Indices=3  OutputSizes=1
  Selector3 : Selector  InputPortWidth=9  IndexOptions=Index vector (dialog)  Indices=4  OutputSizes=1
  Selector4 : Selector  InputPortWidth=9  IndexOptions=Index vector (dialog)  Indices=5  OutputSizes=1
  Selector5 : Selector  InputPortWidth=9  IndexOptions=Index vector (dialog)  Indices=6  OutputSizes=1
  Selector6 : Selector  InputPortWidth=9  IndexOptions=Index vector (dialog)  Indices=7  OutputSizes=1
  Selector7 : Selector  InputPortWidth=9  IndexOptions=Index vector (dialog)  Indices=9  OutputSizes=1
  Selector8 : Selector  InputPortWidth=9  IndexOptions=Index vector (dialog)  Indices=8  OutputSizes=1
  Out1 : Outport
  Out2 : Outport  Port=2
  Out3 : Outport  Port=3
  Out4 : Outport  Port=4
  Out5 : Outport  Port=5
  Out6 : Outport  Port=6
  Out7 : Outport  Port=7
  Out8 : Outport  Port=8
  Out9 : Outport  Port=9
  wires:
  Data Type Conversion3/1 -> Gain3/1
  Selector/1 -> Data Type Conversion/1
  Data Type Conversion7/1 -> Gain7/1
  Sensors/1 -> Selector7/1, Selector8/1, Selector6/1, Selector5/1, Selector1/1, Selector/1, Selector2/1, Selector3/1, Selector4/1  "Sensors"
  Data Type Conversion8/1 -> Gain8/1
  Selector5/1 -> Data Type Conversion5/1
  Data Type Conversion4/1 -> Gain4/1
  Selector3/1 -> Data Type Conversion3/1
  Selector1/1 -> Data Type Conversion1/1
  Data Type Conversion/1 -> Gain/1
  Data Type Conversion6/1 -> Gain6/1
  Selector6/1 -> Data Type Conversion6/1
  Selector7/1 -> Data Type Conversion8/1
  Selector2/1 -> Data Type Conversion2/1
  Data Type Conversion1/1 -> Gain1/1
  Data Type Conversion2/1 -> Gain2/1
  Data Type Conversion5/1 -> Gain5/1
  Selector4/1 -> Data Type Conversion4/1
  Selector8/1 -> Data Type Conversion7/1
  Gain/1 -> Out1/1  "Xpos_m"
  Gain1/1 -> Out2/1  "Xvel_mps"
  Gain2/1 -> Out3/1  "Xacc_mps2"
  Gain3/1 -> Out4/1  "Ypos_m"
  Gain4/1 -> Out5/1  "Yvel_mps"
  Gain5/1 -> Out6/1  "Yacc_mps2"
  Gain6/1 -> Out7/1  "theta_pos_deg"
  Gain7/1 -> Out8/1  "theta_vel_degps"
  Gain8/1 -> Out9/1  "theta_acc_degreeps2"

== system Bossi_Emanuele_EE460S3D_R99/ControlLaw/Observer/InternalObserver/ABM_INT ==
  DX : Inport
  Gain : Gain  Gain=23
  Gain1 : Gain  Gain=16
  Gain2 : Gain  Gain=5
  Product : Product  RndMeth=Zero
  Sum : Sum  Inputs=+-+
  Sum2 : Sum  Inputs=++|
  Unit Delay : UnitDelay  SampleTime=dt  HasFrameUpgradeWarning=on
  Unit Delay1 : UnitDelay  SampleTime=dt  HasFrameUpgradeWarning=on
  Unit Delay2 : UnitDelay  SampleTime=dt  HasFrameUpgradeWarning=on
  dt/12 : Constant  Value=dt/12  SampleTime=dt
  X : Outport
  wires:
  Sum2/1 -> Unit Delay/1
  Product/1 -> Sum2/2
  Unit Delay1/1 -> Gain1/1, Unit Delay2/1
  Gain/1 -> Sum/1
  Gain1/1 -> Sum/2
  Sum/1 -> Product/2
  DX/1 -> Gain/1, Unit Delay1/1
  Unit Delay/1 -> X/1, Sum2/1  "X"
  Gain2/1 -> Sum/3
  Unit Delay2/1 -> Gain2/1
  dt/12/1 -> Product/1

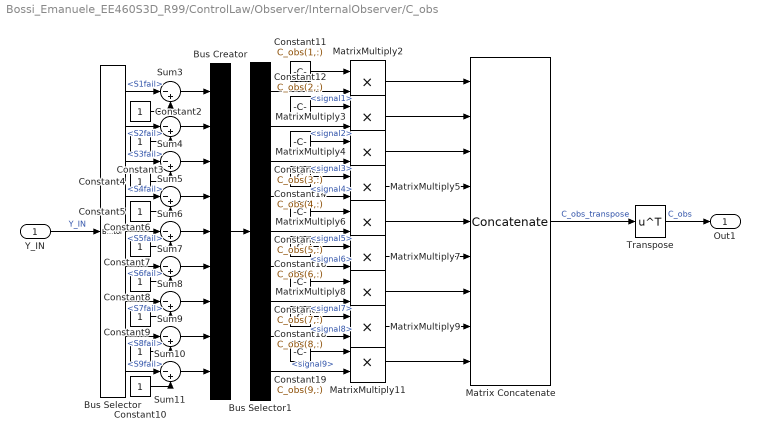
== system Bossi_Emanuele_EE460S3D_R99/ControlLaw/Observer/InternalObserver/C_obs ==
  Y_IN : Inport
  Bus Creator : BusCreator  Inputs=9
  Bus Selector : BusSelector  OutputSignals=S1fail,S2fail,S3fail,S4fail,S5fail,S6fail,S7fail,S8fail,S9fail
  Bus Selector1 : BusSelector  OutputSignals=signal1,signal2,signal3,signal4,signal5,signal6,signal7,signal8,signal9
  Constant{2..10} (9 alike) : Constant
  Constant11 : Constant  Value=C_obs(1,:)
  Constant12 : Constant  Value=C_obs(2,:)
  Constant13 : Constant  Value=C_obs(3,:)
  Constant14 : Constant  Value=C_obs(4,:)
  Constant15 : Constant  Value=C_obs(5,:)
  Constant16 : Constant  Value=C_obs(6,:)
  Constant17 : Constant  Value=C_obs(7,:)
  Constant18 : Constant  Value=C_obs(8,:)
  Constant19 : Constant  Value=C_obs(9,:)
  Matrix Concatenate : Concatenate  NumInputs=9  Mode=Multidimensional array  ConcatenateDimension=2
  MatrixMultiply{2..9,11} (9 alike) : Product
  Sum{3..11} (9 alike) : Sum  Inputs=|-+
  Transpose : Math  Operator=transpose
  Out1 : Outport
  wires:
  Bus Selector1/3 -> MatrixMultiply4/2  "<signal3>"
  Constant12/1 -> MatrixMultiply3/1
  Constant3/1 -> Sum4/2
  Bus Selector1/4 -> MatrixMultiply5/2  "<signal4>"
  Bus Selector/8 -> Sum10/1  "<S8fail>"
  Constant17/1 -> MatrixMultiply8/1
  Constant16/1 -> MatrixMultiply7/1
  Bus Selector1/9 -> MatrixMultiply11/2  "<signal9>"
  Bus Selector1/1 -> MatrixMultiply2/2  "<signal1>"
  Bus Selector1/6 -> MatrixMultiply7/2  "<signal6>"
  Constant10/1 -> Sum11/2
  MatrixMultiply5/1 -> Matrix Concatenate/4
  Constant6/1 -> Sum7/2
  Bus Selector/3 -> Sum5/1  "<S3fail>"
  Sum6/1 -> Bus Creator/4
  Sum11/1 -> Bus Creator/9
  Bus Selector/7 -> Sum9/1  "<S7fail>"
  Sum4/1 -> Bus Creator/2
  Bus Selector/5 -> Sum7/1  "<S5fail>"
  Sum3/1 -> Bus Creator/1
  Bus Selector1/5 -> MatrixMultiply6/2  "<signal5>"
  MatrixMultiply6/1 -> Matrix Concatenate/5
  Constant11/1 -> MatrixMultiply2/1
  Constant18/1 -> MatrixMultiply9/1
  Constant8/1 -> Sum9/2
  MatrixMultiply9/1 -> Matrix Concatenate/8
  MatrixMultiply7/1 -> Matrix Concatenate/6
  Constant14/1 -> MatrixMultiply5/1
  Bus Selector/1 -> Sum3/1  "<S1fail>"
  Constant19/1 -> MatrixMultiply11/1
  MatrixMultiply8/1 -> Matrix Concatenate/7
  Constant5/1 -> Sum6/2
  Bus Selector/9 -> Sum11/1  "<S9fail>"
  Sum10/1 -> Bus Creator/8
  MatrixMultiply11/1 -> Matrix Concatenate/9
  Bus Creator/1 -> Bus Selector1/1
  Constant7/1 -> Sum8/2
  MatrixMultiply3/1 -> Matrix Concatenate/2
  Constant2/1 -> Sum3/2
  Constant9/1 -> Sum10/2
  Y_IN/1 -> Bus Selector/1  "Y_IN"
  Bus Selector/4 -> Sum6/1  "<S4fail>"
  Constant15/1 -> MatrixMultiply6/1
  Sum5/1 -> Bus Creator/3
  Sum7/1 -> Bus Creator/5
  Bus Selector1/8 -> MatrixMultiply9/2  "<signal8>"
  MatrixMultiply4/1 -> Matrix Concatenate/3
  Bus Selector1/2 -> MatrixMultiply3/2  "<signal2>"
  Bus Selector/6 -> Sum8/1  "<S6fail>"
  Constant13/1 -> MatrixMultiply4/1
  MatrixMultiply2/1 -> Matrix Concatenate/1
  Sum8/1 -> Bus Creator/6
  Sum9/1 -> Bus Creator/7
  Bus Selector/2 -> Sum4/1  "<S2fail>"
  Constant4/1 -> Sum5/2
  Bus Selector1/7 -> MatrixMultiply8/2  "<signal7>"
  Matrix Concatenate/1 -> Transpose/1  "C_obs_transpose"
  Transpose/1 -> Out1/1  "C_obs"

== system Bossi_Emanuele_EE460S3D_R99/ControlLaw/Observer/InternalObserver/L ==
  Y_IN : Inport
  Y_IN1 : Inport  Port=2
  In1 : Inport  Port=3
  ABM_INT3 : Subsystem
  C_obs_transpose : Subsystem
  C_obs_transpose1 : Subsystem
  Constant : Constant  Value=G_obs*Q_obs*G_obs'  SampleTime=dt
  Gain1 : Gain  Gain=A_obs  Multiplication=Matrix(K*u)
  Gain2 : Gain  Gain=A_obs'  Multiplication=Matrix(u*K)
  MatrixMultiply{,1..5} (6 alike) : Product  Multiplication=Matrix(*)
  RI : Subsystem
  RI1 : Subsystem
  Sum : Sum  Inputs=|++
  Sum1 : Sum  Inputs=|++
  Sum2 : Sum  Inputs=|+-
  Transpose : Math  Operator=transpose
  Out1 : Outport
  wires:
  Constant/1 -> Sum/1
  Sum/1 -> ABM_INT3/1(DX)  "Pdt"
  Sum1/1 -> Sum/2
  ABM_INT3/1(X) -> MatrixMultiply3/1, MatrixMultiply1/2, MatrixMultiply/1, Gain2/1, Gain1/1  "P"
  Gain1/1 -> Sum1/1
  MatrixMultiply3/1 -> Out1/1
  Sum2/1 -> Sum1/2
  Gain2/1 -> Sum2/1
  MatrixMultiply/1 -> MatrixMultiply1/1
  MatrixMultiply1/1 -> Sum2/2
  Y_IN/1 -> RI/1(Y_IN), C_obs_transpose/1(Y_IN)
  C_obs_transpose/1(Out1) -> MatrixMultiply2/1
  RI/1(Out1) -> MatrixMultiply2/2
  MatrixMultiply2/1 -> MatrixMultiply3/2
  C_obs_transpose1/1(Out1) -> Transpose/1, MatrixMultiply4/1
  RI1/1(Out1) -> MatrixMultiply4/2
  Y_IN1/1 -> C_obs_transpose1/1(Y_IN)
  MatrixMultiply4/1 -> MatrixMultiply5/1
  Transpose/1 -> MatrixMultiply5/2
  MatrixMultiply5/1 -> MatrixMultiply/2
  In1/1 -> RI1/1(Y_IN)

== system Bossi_Emanuele_EE460S3D_R99/ControlLaw/Observer/SensorFailureHandling/Theta ==
  In1 : Inport
  In2 : Inport  Port=2
  In3 : Inport  Port=3
  In4 : Inport  Port=4
  In5 : Inport  Port=5
  In6 : Inport  Port=6
  In7 : Inport  Port=7
  ABM_INT2 : Subsystem
  ABM_INT5 : Subsystem
  Gain2 : Gain  Gain=1/J
  Switch6 : Switch  Criteria=u2 > Threshold  SaturateOnIntegerOverflow=off  InputSameDT=off
  Switch7 : Switch  Criteria=u2 > Threshold  SaturateOnIntegerOverflow=off  InputSameDT=off
  Switch8 : Switch  Criteria=u2 > Threshold  SaturateOnIntegerOverflow=off  InputSameDT=off
  Out1 : Outport
  Out2 : Outport  Port=2
  Out3 : Outport  Port=3
  wires:
  Switch6/1 -> Out1/1, ABM_INT5/1(DX)  "theta_acc_degreeps2"
  In5/1 -> Switch7/3
  In4/1 -> Switch7/2
  Gain2/1 -> Switch6/1
  In2/1 -> Switch6/2
  ABM_INT2/1(X) -> Switch8/1  "X_hat"
  In1/1 -> Gain2/1
  ABM_INT5/1(X) -> Switch7/1  "X_hat"
  In6/1 -> Switch8/2
  In7/1 -> Switch8/3
  In3/1 -> Switch6/3
  Switch8/1 -> Out3/1  "theta_pos_deg"
  Switch7/1 -> Out2/1, ABM_INT2/1(DX)  "theta_vel_degps"

== system Bossi_Emanuele_EE460S3D_R99/ControlLaw/Observer/SensorFailureHandling/X ==
  In1 : Inport
  In2 : Inport  Port=2
  In3 : Inport  Port=3
  In4 : Inport  Port=4
  In5 : Inport  Port=5
  In6 : Inport  Port=6
  In7 : Inport  Port=7
  ABM_INT : Subsystem
  ABM_INT3 : Subsystem
  Gain : Gain  Gain=1/M
  Switch : Switch  Criteria=u2 > Threshold  SaturateOnIntegerOverflow=off  InputSameDT=off
  Switch1 : Switch  Criteria=u2 > Threshold  SaturateOnIntegerOverflow=off  InputSameDT=off
  Switch2 : Switch  Criteria=u2 > Threshold  SaturateOnIntegerOverflow=off  InputSameDT=off
  Out1 : Outport
  Out2 : Outport  Port=2
  Out3 : Outport  Port=3
  wires:
  In1/1 -> Gain/1
  In2/1 -> Switch/2
  In5/1 -> Switch1/3
  In7/1 -> Switch2/3
  Switch/1 -> Out1/1, ABM_INT3/1(DX)  "Xacc_mps2"
  Switch1/1 -> Out2/1, ABM_INT/1(DX)  "Xvel_mps"
  Switch2/1 -> Out3/1  "Xpos_m"
  Gain/1 -> Switch/1
  In3/1 -> Switch/3
  ABM_INT3/1(X) -> Switch1/1  "X_hat"
  ABM_INT/1(X) -> Switch2/1  "X_hat"
  In4/1 -> Switch1/2
  In6/1 -> Switch2/2

== system Bossi_Emanuele_EE460S3D_R99/ControlLaw/Observer/SensorFailureHandling/Y ==
  In1 : Inport
  In2 : Inport  Port=2
  In3 : Inport  Port=3
  In4 : Inport  Port=4
  In5 : Inport  Port=5
  In6 : Inport  Port=6
  In7 : Inport  Port=7
  ABM_INT1 : Subsystem
  ABM_INT4 : Subsystem
  Gain1 : Gain  Gain=1/M
  Switch3 : Switch  Criteria=u2 > Threshold  SaturateOnIntegerOverflow=off  InputSameDT=off
  Switch4 : Switch  Criteria=u2 > Threshold  SaturateOnIntegerOverflow=off  InputSameDT=off
  Switch5 : Switch  Criteria=u2 > Threshold  SaturateOnIntegerOverflow=off  InputSameDT=off
  Out1 : Outport
  Out2 : Outport  Port=2
  Out3 : Outport  Port=3
  wires:
  In3/1 -> Switch3/3
  ABM_INT4/1(X) -> Switch4/1  "X_hat"
  In4/1 -> Switch4/2
  ABM_INT1/1(X) -> Switch5/1  "X_hat"
  In7/1 -> Switch5/3
  In1/1 -> Gain1/1
  In6/1 -> Switch5/2
  In5/1 -> Switch4/3
  Gain1/1 -> Switch3/1
  In2/1 -> Switch3/2
  Switch3/1 -> Out1/1, ABM_INT4/1(DX)  "Yacc_mps2"
  Switch5/1 -> Out3/1  "Ypos_m"
  Switch4/1 -> Out2/1, ABM_INT1/1(DX)  "Yvel_mps"
